simulink model "pi_speed_control_dc_machine_block"  (R2024b)
settings: Solver=VariableStepAuto  StartTime=0.0  StopTime=2  RelTol=1e-3
undefined symbols (not defined in the file): J_m, kfi, L_a, R_a, T_n
libraries: spsControlledVoltageSourceLib x4, spsDCMachineLib x4, spspowerguiLib x3, sps_lib x1
settings Model: Creator=SCH 2  LastModifiedBy=DE MK HU
settings DebuggingCC: UnderspecifiedInitializationDetection=Classic  MergeDetectMultiDrivingBlocksExec=none
settings ModelReferenceCC: PropagateSignalLabelsOutOfModel=off

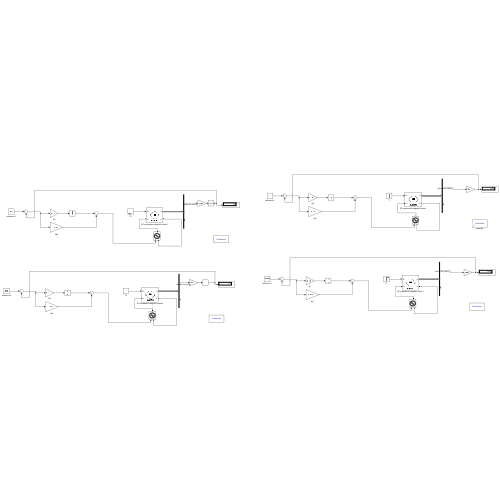
[thumbnail: Simulink's stored preview of the top-level diagram]
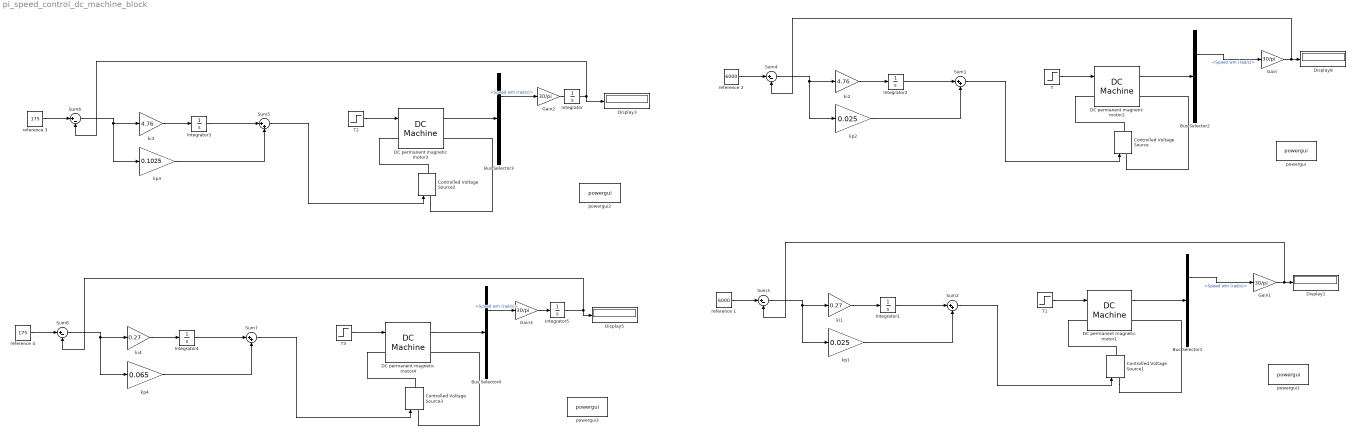
== system pi_speed_control_dc_machine_block ==
  Bus Selector{1..4} (4 alike) : BusSelector  OutputSignals=Speed wm (rad/s),Armature current ia (A)
  Controlled Voltage Source{,1..3} (4 alike) : spsControlledVoltageSourceLib/Controlled Voltage Source  Initialize=on  Source_Type=AC  Amplitude=0  Phase=0  Frequency=0  Measurements=None
  DC permanent magnetic motor{1..4} (4 alike) : spsDCMachineLib/DC Machine  PresetModel=No  MechanicalLoad=Torque TL  FieldType=Permanent magnet  ShowDetailedParameters=on  MeasurementBus=off  RLa=[R_a L_a]  RLf=[180 71.47]  Laf=1.345  MachineConstant=Torque constant (N.m/A)  Ke=1.8  Kt=kfi  J=J_m  Bm=B_m  Tf=0  w0=1340.413  Ifinit=1  TsPowergui=0  TsBlock=-1
  Display{1,3,5,8} (4 alike) : Display
  Gain{,1..3} (4 alike) : Gain  Gain=30/pi
  Integrator{,1..5} (6 alike) : Integrator
  Sum{1..2,5,7} (4 alike) : Sum  Inputs=|++
  Sum{3..4,6,8} (4 alike) : Sum  Inputs=|+-
  T{,1..3} (4 alike) : Step  Time=2  After=T_n  SampleTime=0
  ki1 : Gain  Gain=0.27
  ki2 : Gain  Gain=4.76
  ki3 : Gain  Gain=4.76
  ki4 : Gain  Gain=0.27
  kp1 : Gain  Gain=0.025
  kp2 : Gain  Gain=0.025
  kp3 : Gain  Gain=0.1025
  kp4 : Gain  Gain=0.065
  powergui : sps_lib/powergui  Priority=1  SimulationMode=Continuous  SampleTime=50e-6  frequency=60  Iterations=50  frequencyindice=0  Pbase=100e6  ErrMax=1e-4  UnitsV=kV  UnitsW=MW  buscounter=0  FunctionMessages=off  echomessages=off  EnableUseOfTLC=off  CurrentSourceSwitches=off  DisableSnubberDevices=off  DisableRonSwitches=off  DisableVfSwitches=off  DisplayEquations=off  AutomaticDiscreteSolvers=off  SolverType=Tustin/Backward Euler (TBE)  Interpol=off  ExternalGateDelay=off  methode=off  Ts=100  x0status=blocks  SPID=on  SwTol=0  HookPort=off  NonlinearTolerance=1e-4  nMaxIteration=100  ContinueOnMaxIteration=off  RestoreLinks=warning  ResistiveCurrentMeasurement=off  Frange=[0:2:500]  Ylog=off  Xlog=on  ShowGrid=off  save=off  variable=ZData  structure=0  ZoomFFT=off  StartTime=0.0  cycles=1  DisplayStyle=1  fundamental=60  FreqAxis=off  MaxFrequency=1000  frequencyindicesteady=1  RmsSteady=1  display=off
  powergui1 : spspowerguiLib/powergui  Priority=1  SimulationMode=Continuous  SampleTime=50e-6  frequency=60  Iterations=50  frequencyindice=0  Pbase=100e6  ErrMax=1e-4  UnitsV=kV  UnitsW=MW  buscounter=0  FunctionMessages=off  echomessages=off  EnableUseOfTLC=off  CurrentSourceSwitches=off  DisableSnubberDevices=off  DisableRonSwitches=off  DisableVfSwitches=off  DisplayEquations=off  AutomaticDiscreteSolvers=off  SolverType=Tustin/Backward Euler (TBE)  Interpol=off  ExternalGateDelay=off  methode=off  Ts=100  x0status=blocks  SPID=on  SwTol=0  HookPort=off  NonlinearTolerance=1e-4  nMaxIteration=100  ContinueOnMaxIteration=off  RestoreLinks=warning  ResistiveCurrentMeasurement=off  Frange=[0:2:500]  Ylog=off  Xlog=on  ShowGrid=off  save=off  variable=ZData  structure=0  ZoomFFT=off  StartTime=0.0  cycles=1  DisplayStyle=1  fundamental=60  FreqAxis=off  MaxFrequency=1000  frequencyindicesteady=1  RmsSteady=1  display=off
  powergui2 : spspowerguiLib/powergui  Priority=1  SimulationMode=Continuous  SampleTime=50e-6  frequency=60  Iterations=50  frequencyindice=0  Pbase=100e6  ErrMax=1e-4  UnitsV=kV  UnitsW=MW  buscounter=0  FunctionMessages=off  echomessages=off  EnableUseOfTLC=off  CurrentSourceSwitches=off  DisableSnubberDevices=off  DisableRonSwitches=off  DisableVfSwitches=off  DisplayEquations=off  AutomaticDiscreteSolvers=off  SolverType=Tustin/Backward Euler (TBE)  Interpol=off  ExternalGateDelay=off  methode=off  Ts=100  x0status=blocks  SPID=on  SwTol=0  HookPort=off  NonlinearTolerance=1e-4  nMaxIteration=100  ContinueOnMaxIteration=off  RestoreLinks=warning  ResistiveCurrentMeasurement=off  Frange=[0:2:500]  Ylog=off  Xlog=on  ShowGrid=off  save=off  variable=ZData  structure=0  ZoomFFT=off  StartTime=0.0  cycles=1  DisplayStyle=1  fundamental=60  FreqAxis=off  MaxFrequency=1000  frequencyindicesteady=1  RmsSteady=1  display=off
  powergui3 : spspowerguiLib/powergui  Priority=1  SimulationMode=Continuous  SampleTime=50e-6  frequency=60  Iterations=50  frequencyindice=0  Pbase=100e6  ErrMax=1e-4  UnitsV=kV  UnitsW=MW  buscounter=0  FunctionMessages=off  echomessages=off  EnableUseOfTLC=off  CurrentSourceSwitches=off  DisableSnubberDevices=off  DisableRonSwitches=off  DisableVfSwitches=off  DisplayEquations=off  AutomaticDiscreteSolvers=off  SolverType=Tustin/Backward Euler (TBE)  Interpol=off  ExternalGateDelay=off  methode=off  Ts=100  x0status=blocks  SPID=on  SwTol=0  HookPort=off  NonlinearTolerance=1e-4  nMaxIteration=100  ContinueOnMaxIteration=off  RestoreLinks=warning  ResistiveCurrentMeasurement=off  Frange=[0:2:500]  Ylog=off  Xlog=on  ShowGrid=off  save=off  variable=ZData  structure=0  ZoomFFT=off  StartTime=0.0  cycles=1  DisplayStyle=1  fundamental=60  FreqAxis=off  MaxFrequency=1000  frequencyindicesteady=1  RmsSteady=1  display=off
  reference 1 : Constant  Value=6000
  reference 2 : Constant  Value=6000
  reference 3 : Constant  Value=175
  reference 4 : Constant  Value=175
  wires:
  T/1 -> DC permanent magnetic motor2/1
  DC permanent magnetic motor2/1 -> Bus Selector2/1
  Bus Selector2/1 -> Gain/1  "<Speed wm (rad/s)>"
  Gain/1 -> Sum4/2, Display8/1
  Sum4/1 -> kp2/1, ki2/1
  reference 2/1 -> Sum4/1
  Integrator2/1 -> Sum1/1
  kp2/1 -> Sum1/2
  ki2/1 -> Integrator2/1
  Sum1/1 -> Controlled Voltage Source/1
  kp1/1 -> Sum2/2
  Integrator1/1 -> Sum2/1
  reference 1/1 -> Sum3/1
  Sum3/1 -> kp1/1, ki1/1
  Bus Selector1/1 -> Gain1/1  "<Speed wm (rad/s)>"
  T1/1 -> DC permanent magnetic motor1/1
  ki1/1 -> Integrator1/1
  DC permanent magnetic motor1/1 -> Bus Selector1/1
  Gain1/1 -> Sum3/2, Display1/1
  Sum2/1 -> Controlled Voltage Source1/1
  kp3/1 -> Sum5/2
  Integrator3/1 -> Sum5/1
  reference 3/1 -> Sum6/1
  Sum6/1 -> kp3/1, ki3/1
  Bus Selector3/1 -> Gain2/1  "<Speed wm (rad/s)>"
  T2/1 -> DC permanent magnetic motor3/1
  ki3/1 -> Integrator3/1
  DC permanent magnetic motor3/1 -> Bus Selector3/1
  Gain2/1 -> Display3/1, Sum6/2
  Sum5/1 -> Controlled Voltage Source2/1
  kp4/1 -> Sum7/2
  Integrator4/1 -> Sum7/1
  reference 4/1 -> Sum8/1
  Sum8/1 -> kp4/1, ki4/1
  Bus Selector4/1 -> Gain3/1  "<Speed wm (rad/s)>"
  T3/1 -> DC permanent magnetic motor4/1
  ki4/1 -> Integrator4/1
  DC permanent magnetic motor4/1 -> Bus Selector4/1
  Gain3/1 -> Integrator5/1
  Sum7/1 -> Controlled Voltage Source3/1
  Integrator5/1 -> Display5/1, Sum8/2
  connections:
  Controlled Voltage Source/RConn1 -- DC permanent magnetic motor2/LConn1
  Controlled Voltage Source/LConn1 -- DC permanent magnetic motor2/RConn1
  Controlled Voltage Source1/RConn1 -- DC permanent magnetic motor1/LConn1
  Controlled Voltage Source1/LConn1 -- DC permanent magnetic motor1/RConn1
  Controlled Voltage Source2/RConn1 -- DC permanent magnetic motor3/LConn1
  Controlled Voltage Source2/LConn1 -- DC permanent magnetic motor3/RConn1
  Controlled Voltage Source3/RConn1 -- DC permanent magnetic motor4/LConn1
  Controlled Voltage Source3/LConn1 -- DC permanent magnetic motor4/RConn1
